simulink model "DC_Motor_FOPID"  (R2026b)
settings: Solver=VariableStepAuto
settings Model: Creator=Shobhit  LastModifiedBy=Shobhit

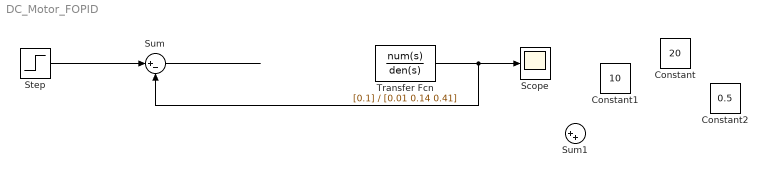
== system DC_Motor_FOPID ==
  Constant : Constant  Value=20
  Constant1 : Constant  Value=10
  Constant2 : Constant  Value=0.5
  Scope : Scope
      settings: ActiveDisplayYMinimum=-0.12500699060955561  ActiveDisplayYMaximum=1.1250629154860008
  Step : Step  Time=0  SampleTime=0
  Sum : Sum  Inputs=|+-
  Sum1 : Sum  Inputs=|++
  Transfer Fcn : TransferFcn  Numerator=[0.1]  Denominator=[0.01 0.14 0.41]
  wires:
  Step/1 -> Sum/1
  Sum/1 -> ?
  ? -> Transfer Fcn/1
  Transfer Fcn/1 -> Sum/2, Scope/1
